simulink model "sm_wheel_loader"  (R2025a)
settings: Solver=ode23t  StartTime=0.0  StopTime=70  RelTol=1e-3  AbsTol=1e-3  EnableMultiTasking=on
PostLoadFcn:
  | sm_wheel_loader_config_impl(bdroot,'Bucket')
StartFcn:
  | tic
StopFcn:
  | Elapsed_Sim_Time = toc;
  | disp(['Elapsed Sim Time = ' num2str(Elapsed_Sim_Time)]);
undefined symbols (not defined in the file or in its folder): HMPST, Ideal, X, Y, Z
libraries: sm_wheel_loader_lib x9, fl_lib x4, sm_lib x3, sdl_lib x2, wheel_loader_contact_lib x2, nesl_utility x1
Description:
  | Wheel Loader with Hydromechanical Power Split Transmission
  | Copyright 2023-2025 The MathWorks, Inc.
settings Model: Creator=ramesh  LastModifiedBy=smiller
settings ConfigSet: Description=|
  | This is the default simulation configuration set.
  | This configuration is used for simulating the model for IK, RBD simulations.
  | This uses variable-step solver.
settings SolverCC: AutoScaleAbsTol=off  AlgebraicLoopSolver=TrustRegion  DecoupledContinuousIntegration=on  MinimalZcImpactIntegration=on
settings DataIOCC: MaxDataPoints=10000  DSMLogging=off  ReturnWorkspaceOutputs=off  SignalLoggingName=logsout_sm_wheel_loader  OutputTimes=[0:0.01:stopTime]
settings OptimizationCC: LifeSpan=inf
settings DebuggingCC: UnconnectedInputMsg=warning  UnconnectedOutputMsg=warning  UnconnectedLineMsg=warning  AllowSymbolicDim=off  SFUnexpectedBacktrackingDiag=warning  SFNoUnconditionalDefaultTransitionDiag=warning  SFExecutionAtInitializationDiag=none  ArithmeticOperatorsInVariantConditions=warning
settings ModelReferenceCC: EnableRefExpFcnMdlSchedulingChecks=on
settings SFSimCC: SimUseLocalCustomCode=off  CustomCodeUndefinedFunction=UseInterfaceOnly
settings RTWCC: RTWUseLocalCustomCode=off  GPUComputeCapability=3.5  DLArmComputeVersion=19.05
settings CodeAppCC: StateflowObjectComments=on
settings GRTTargetCC: TargetLangStandard=C89/C90 (ANSI)
settings ConfigComp: CovMetricSettings=dw  CovSaveCumulativeToWorkspaceVar=on  CovSaveSingleToWorkspaceVar=on  CovExternalEMLEnable=off  CovSFcnEnable=off
settings SimscapeCC: SimscapeLogType=all  SimscapeLogSimulationStatistics=on  SimscapeLogName=simlog_sm_wheel_loader  SimscapeLogLimitData=off  SimscapeLogDataHistory=10000.0
settings DiagnosticsConfigSet: SimMechanicsUnconnectedFramePorts=none  SimMechanicsConflictingReferenceFrames=none
settings ExplorerConfigSet: InternalSimMechanicsExplorerSettings="<ExplorerConfiguration><canonicalview>default</canonicalview><AnimationSetting><BasePlaybackSpeed>1.0</BasePlaybackSpeed><PlaybackSpeedFactor>4.0</PlaybackSpeedFactor></AnimationSetting><TilePanel><TileInfo><Tiles Columns=\"2\" Count=\"3\" Rows=\"2\"><Column Weight=\"0.5\"/><Column Weight=\"0.5\"/><Row Weight=\"0.5\"/><Row Weight=\"0.5\"/><Tile Height=\"2\" Width=\"1\" X=\"0\" Y=\"0\"/><Tile Height=\"1\" Width=\"1\" X=\"1\" Y=\"0\"/><Tile Height=\"1\" Width=\"1\" X=\"1\" Y=\"1\"/></Tiles></TileInfo><SceneInfo><SceneViewer><BGColor><R>1</R><G>1</G><B>1</B></BGColor><Camera><DoPerspective>off</DoPerspective><Position><X>-0.00528186565900144213</X><Y>-2.61761552453344981</Y><Z>10.0638099418932807</Z></Position><Center><X>-0.00528186565900144213</X><Y>-2.61761552453344981</Y><Z>1.2817155600129837</Z></Center><Up><X>0</X><Y>1</Y><Z>-0</Z></Up><ViewLimDist>1</ViewLimDist><YLim>8.29414102564102684</YLim><XLim>9.06400000000000006</XLim></Camera></SceneViewer><SceneViewer><BGColor><R>1</R><G>1</G><B>1</B></BGColor><Camera><DoPerspective>on</DoPerspective><Position><X>1.34928960365821002e-16</X><Y>1.6204999999999985</Y><Z>1.58342999999999989</Z></Position><Center><X>8.83082669489443361e-17</X><Y>0.620499999999998497</Y><Z>1.58343000000000012</Z></Center><Up><X>0</X><Y>0</Y><Z>1</Z></Up><ViewLimDist>1</ViewLimDist><YLim>0.466307658154998583</YLim><XLim>1.0355017035185734</XLim></Camera></SceneViewer><SceneViewer><BGColor><R>1</R><G>1</G><B>1</B></BGColor><Camera><DoPerspective>on</DoPerspective><Position><X>-4.09999999999999964</X><Y>-0.0795000000000013474</Y><Z>1.08343000000000012</Z></Position><Center><X>-3.09999999999999964</X><Y>-0.079500000000001389</Y><Z>1.08343000000000012</Z></Center><Up><X>0</X><Y>0</Y><Z>1</Z></Up><ViewLimDist>1</ViewLimDist><YLim>0.466307658154998583</YLim><XLim>1.0355017035185734</XLim></Camera></SceneViewer></SceneInfo></TilePanel><MechEditorPanel><Cameras><Camera><Id>Camera2</Id><Value><Name>Track_FrameR_DiffR_toR</Name><NativeCamera><PositionTrackingFeature>Wheel_Loader.Vehicle.Frame_Rear.Camera_Frames.Reference_Camera_DiffR_toR.R</PositionTrackingFeature><CenterTrackingFeature>Wheel_Loader.Vehicle.Frame_Rear.Camera_Frames.Reference_Camera_DiffR_toR.R</CenterTrackingFeature><UpVectorTrackingFeature>Wheel_Loader.Vehicle.Frame_Rear.Camera_Frames.Reference_Camera_DiffR_toR.R</UpVectorTrackingFeature><CenterTrackingOrigin>off</CenterTrackingOrigin><CenterTrackingDirection>-Y</CenterTrackingDirection><UpVectorTrackingDirection>+Z</UpVectorTrackingDirection></NativeCamera></Value></Camera><Camera><Id>Camera3</Id><Value><Name>Track_FrameR_FinalDriveRR</Name><NativeCamera><PositionTrackingFeature>Wheel_Loader.Vehicle.Frame_Rear.Camera_Frames.Reference_Camera_FinalDriveRR.R</PositionTrackingFeature><CenterTrackingFeature>Wheel_Loader.Vehicle.Frame_Rear.Camera_Frames.Reference_Camera_FinalDriveRR.R</CenterTrackingFeature><UpVectorTrackingFeature>Wheel_Loader.Vehicle.Frame_Rear.Camera_Frames.Reference_Camera_FinalDriveRR.R</UpVectorTrackingFeature><CenterTrackingOrigin>off</CenterTrackingOrigin><CenterTrackingDirection>-X</CenterTrackingDirection><UpVectorTrackingDirection>+Z</UpVectorTrackingDirection></NativeCamera></Value></Camera><Camera><Id>Camera4</Id><Value><Name>Track_FrameR_Right</Name><NativeCamera><PositionTrackingFeature>Wheel_Loader.Vehicle.Frame_Rear.Camera_Frames.Reference_Camera_Right.R</PositionTrackingFeature><CenterTrackingFeature>Wheel_Loader.Vehicle.Frame_Rear.Camera_Frames.Reference_Camera_Right.R</CenterTrackingFeature><UpVectorTrackingFeature>Wheel_Loader.World_Frame.W</UpVectorTrackingFeature><CenterTrackingOrigin>off</CenterTrackingOrigin><CenterTrackingDirection>-X</CenterTrackingDirection><UpVectorTrackingDirection>+Z</UpVectorTrackingDirection></NativeCamera></Value></Camera><Camera><Id>Camera5</Id><Value><Name>Track_FrameR_Cab</Name><NativeCamera><PositionTrackingFeature>Wheel_Loader.Vehicle.Frame_Rear.Camera_Frames.Reference_Camera_Cab.R</PositionTrackingFeature><CenterTrackingFeature>Wheel_Loader.Vehicle.Frame_Rear.Camera_Frames.Reference_Camera_Cab.R</CenterTrackingFeature><UpVectorTrackingFeature>Wheel_Loader.World_Frame.W</UpVectorTrackingFeature><CenterTrackingOrigin>off</CenterTrackingOrigin><CenterTrackingDirection>+Y</CenterTrackingDirection><UpVectorTrackingDirection>+Z</UpVectorTrackingDirection></NativeCamera></Value></Camera><Camera><Id>Camera6</Id><Value><Name>Track_FrameR_RR</Name><NativeCamera><PositionTrackingFeature>Wheel_Loader.Vehicle.Frame_Rear.Camera_Frames.Reference_Camera_RR.R</PositionTrackingFeature><CenterTrackingFeature>Wheel_Loader.Vehicle.Frame_Rear.Camera_Frames.Reference_Camera_RR.R</CenterTrackingFeature><UpVectorTrackingFeature>Wheel_Loader.World_Frame.W</UpVectorTrackingFeature><CenterTrackingOrigin>off</CenterTrackingOrigin><CenterTrackingDirection>+X</CenterTrackingDirection><UpVectorTrackingDirection>+Z</UpVectorTrackingDirection></NativeCamera></Value></Camera><Camera><Id>Camera7</Id><Value><Name>Track_FrameR_Rear</Name><NativeCamera><PositionTrackingFeature>Wheel_Loader.Vehicle.Frame_Rear.Camera_Frames.Reference_Camera_Rear.R</PositionTrackingFeature><CenterTrackingFeature>Wheel_Loader.Vehicle.Frame_Rear.Camera_Frames.Reference_Camera_Rear.R</CenterTrackingFeature><UpVectorTrackingFeature>Wheel_Loader.World_Frame.W</UpVectorTrackingFeature><CenterTrackingOrigin>off</CenterTrackingOrigin><CenterTrackingDirection>+Y</CenterTrackingDirection><UpVectorTrackingDirection>+Z</UpVectorTrackingDirection></NativeCamera></Value></Camera><Camera><Id>Camera8</Id><Value><Name>Track_FrameF_RR</Name><NativeCamera><PositionTrackingFeature>Wheel_Loader.Vehicle.Frame_Front.Camera_Frames.Reference_Camera_RR.R</PositionTrackingFeature><CenterTrackingFeature>Wheel_Loader.Vehicle.Frame_Front.Camera_Frames.Reference_Camera_RR.R</CenterTrackingFeature><UpVectorTrackingFeature>Wheel_Loader.Vehicle.Frame_Front.Camera_Frames.Reference_Camera_RR.R</UpVectorTrackingFeature><CenterTrackingOrigin>off</CenterTrackingOrigin><CenterTrackingDirection>+X</CenterTrackingDirection><UpVectorTrackingDirection>+Z</UpVectorTrackingDirection></NativeCamera></Value></Camera><Camera><Id>Camera9</Id><Value><Name>Track_FrameF_ImplRR</Name><NativeCamera><PositionTrackingFeature>Wheel_Loader.Vehicle.Frame_Front.Camera_Frames.Reference_Camera_ImplRR.R</PositionTrackingFeature><CenterTrackingFeature>Wheel_Loader.Vehicle.Frame_Front.Camera_Frames.Reference_Camera_ImplRR.R</CenterTrackingFeature><UpVectorTrackingFeature>Wheel_Loader.Vehicle.Frame_Front.Camera_Frames.Reference_Camera_ImplRR.R</UpVectorTrackingFeature><CenterTrackingOrigin>off</CenterTrackingOrigin><CenterTrackingDirection>+X</CenterTrackingDirection><UpVectorTrackingDirection>+Z</UpVectorTrackingDirection></NativeCamera></Value></Camera><Camera><Id>Camera10</Id><Value><Name>Track_FrameF_Roof</Name><NativeCamera><PositionTrackingFeature>Wheel_Loader.Vehicle.Frame_Front.Camera_Frames.Reference_Camera_Roof.R</PositionTrackingFeature><CenterTrackingFeature>Wheel_Loader.Vehicle.Frame_Front.Camera_Frames.Reference_Camera_Roof.R</CenterTrackingFeature><UpVectorTrackingFeature>Wheel_Loader.Vehicle.Frame_Front.Camera_Frames.Reference_Camera_Roof.R</UpVectorTrackingFeature><CenterTrackingOrigin>off</CenterTrackingOrigin><CenterTrackingDirection>+Y</CenterTrackingDirection><UpVectorTrackingDirection>+Z</UpVectorTrackingDirection></NativeCamera></Value></Camera><Camera><Id>Camera11</Id><Value><Name>Track_FrameR_Driveline_RR</Name><NativeCamera><PositionTrackingFeature>Wheel_Loader.Vehicle.Frame_Rear.Camera_Frames.Reference_Camera_Driveline_RR.R</PositionTrackingFeature><CenterTrackingFeature>Wheel_Loader.Vehicle.Frame_Rear.Camera_Frames.Reference_Camera_Driveline_RR.R</CenterTrackingFeature><UpVectorTrackingFeature>Wheel_Loader.Vehicle.Frame_Rear.Camera_Frames.Reference_Camera_Driveline_RR.R</UpVectorTrackingFeature><CenterTrackingOrigin>off</CenterTrackingOrigin><CenterTrackingDirection>+Y</CenterTrackingDirection><UpVectorTrackingDirection>+Z</UpVectorTrackingDirection></NativeCamera></Value></Camera><Camera><Id>Camera12</Id><Value><Name>Track_FrameR_Driveline_Top</Name><NativeCamera><PositionTrackingFeature>Wheel_Loader.Vehicle.Frame_Rear.Camera_Frames.Reference_Camera_Driveline_Top.R</PositionTrackingFeature><CenterTrackingFeature>Wheel_Loader.Vehicle.Frame_Rear.Camera_Frames.Reference_Camera_Driveline_Top.R</CenterTrackingFeature><UpVectorTrackingFeature>Wheel_Loader.Vehicle.Frame_Rear.Camera_Frames.Reference_Camera_Driveline_Top.R</UpVectorTrackingFeature><CenterTrackingOrigin>off</CenterTrackingOrigin><CenterTrackingDirection>-Z</CenterTrackingDirection><UpVectorTrackingDirection>-X</UpVectorTrackingDirection></NativeCamera></Value></Camera><Camera><Id>Camera13</Id><Value><Name>Track_FrameR_Driveline_Top_FixO</Name><NativeCamera><PositionTrackingFeature>Wheel_Loader.Vehicle.Frame_Rear.Camera_Frames.Reference_Camera_Driveline_Top.R</PositionTrackingFeature><CenterTrackingFeature>Wheel_Loader.Vehicle.Frame_Rear.Camera_Frames.Reference_Camera_Driveline_Top.R</CenterTrackingFeature><UpVectorTrackingFeature>Wheel_Loader.World_Frame.W</UpVectorTrackingFeature><CenterTrackingOrigin>off</CenterTrackingOrigin><CenterTrackingDirection>-Z</CenterTrackingDirection><UpVectorTrackingDirection>+X</UpVectorTrackingDirection></NativeCamera></Value></Camera><Camera><Id>Camera14</Id><Value><Name>Track_FrameR_DiffR_toF</Name><NativeCamera><PositionTrackingFeature>Wheel_Loader.Vehicle.Frame_Rear.Camera_Frames.Reference_Camera_DiffR_toF.R</PositionTrackingFeature><CenterTrackingFeature>Wheel_Loader.Vehicle.Frame_Rear.Camera_Frames.Reference_Camera_DiffR_toF.R</CenterTrackingFeature><UpVectorTrackingFeature>Wheel_Loader.Vehicle.Frame_Rear.Camera_Frames.Reference_Camera_DiffR_toF.R</UpVectorTrackingFeature><CenterTrackingOrigin>off</CenterTrackingOrigin><CenterTrackingDirection>-Y</CenterTrackingDirection><UpVectorTrackingDirection>+Z</UpVectorTrackingDirection></NativeCamera></Value></Camera><Camera><Id>Camera15</Id><Value><Name>Track_FrameR_Driveline_Top_Low</Name><NativeCamera><PositionTrackingFeature>Wheel_Loader.Vehicle.Frame_Rear.Camera_Frames.Reference_Camera_Driveline_TopLow.R</PositionTrackingFeature><CenterTrackingFeature>Wheel_Loader.Vehicle.Frame_Rear.Camera_Frames.Reference_Camera_Driveline_TopLow.R</CenterTrackingFeature><UpVectorTrackingFeature>Wheel_Loader.Vehicle.Frame_Rear.Camera_Frames.Reference_Camera_Driveline_TopLow.R</UpVectorTrackingFeature><CenterTrackingOrigin>off</CenterTrackingOrigin><CenterTrackingDirection>-Z</CenterTrackingDirection><UpVectorTrackingDirection>-X</UpVectorTrackingDirection></NativeCamera></Value></Camera><Camera><Id>Camera16</Id><Value><Name>Track_FrameF_LinkageR</Name><NativeCamera><PositionTrackingFeature>Wheel_Loader.Vehicle.Frame_Front.Camera_Frames.Transform_Camera_LinkageR.F</PositionTrackingFeature><CenterTrackingFeature>Wheel_Loader.Vehicle.Frame_Front.Camera_Frames.Transform_Camera_LinkageR.F</CenterTrackingFeature><UpVectorTrackingFeature>Wheel_Loader.Vehicle.Frame_Front.Camera_Frames.Transform_Camera_LinkageR.F</UpVectorTrackingFeature><CenterTrackingOrigin>off</CenterTrackingOrigin><CenterTrackingDirection>-X</CenterTrackingDirection><UpVectorTrackingDirection>+Z</UpVectorTrackingDirection></NativeCamera></Value></Camera><Camera><Id>Camera17</Id><Value><Name>TrackF_WheelFR</Name><NativeCamera><PositionTrackingFeature>Wheel_Loader.Vehicle.Frame_Front.Camera_Frames.Reference_Camera_WhlFR.R</PositionTrackingFeature><CenterTrackingFeature>Wheel_Loader.Vehicle.Frame_Front.Camera_Frames.Reference_Camera_WhlFR.R</CenterTrackingFeature><UpVectorTrackingFeature>Wheel_Loader.World_Frame.W</UpVectorTrackingFeature><CenterTrackingOrigin>off</CenterTrackingOrigin><CenterTrackingDirection>-X</CenterTrackingDirection><UpVectorTrackingDirection>+Z</UpVectorTrackingDirection></NativeCamera></Value></Camera><Camera><Id>Camera18</Id><Value><Name>TrackF_IsoFR</Name><NativeCamera><PositionTrackingFeature>Wheel_Loader.Vehicle.Frame_Front.Camera_Frames.Reference_Camera_IsoFR.R</PositionTrackingFeature><CenterTrackingFeature>Wheel_Loader.Vehicle.Frame_Front.Camera_Frames.Reference_Camera_IsoFR.R</CenterTrackingFeature><UpVectorTrackingFeature>Wheel_Loader.World_Frame.W</UpVectorTrackingFeature><CenterTrackingOrigin>off</CenterTrackingOrigin><CenterTrackingDirection>-X</CenterTrackingDirection><UpVectorTrackingDirection>+Z</UpVectorTrackingDirection></NativeCamera></Value></Camera></Cameras><GfxPanelCameraMap><MapElement CameraMLId=\"Camera5\" GfxPanelIndex=\"1\"/><MapElement CameraMLId=\"Camera4\" GfxPanelIndex=\"2\"/></GfxPanelCameraMap><VideoCreator><PlaybackSpeedRatio>1</PlaybackSpeedRatio><FrameRate>30</FrameRate><VideoFormat>MPEG-4</VideoFormat><FrameSize>auto</FrameSize></VideoCreator></MechEditorPanel></ExplorerConfiguration>"

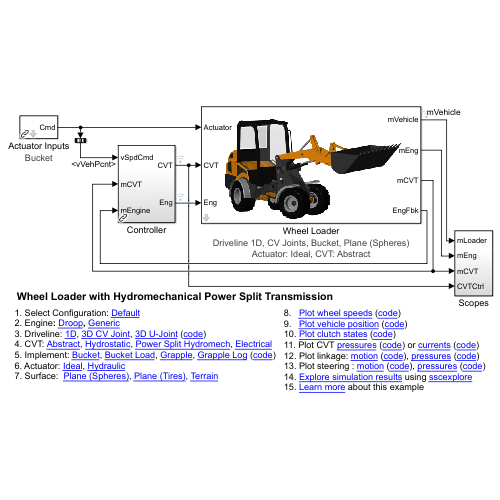
[thumbnail: Simulink's stored preview of the top-level diagram]
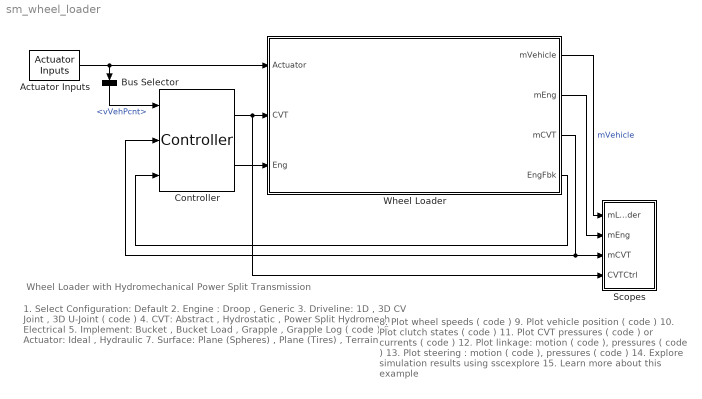
== system sm_wheel_loader ==
  note: Wheel Loader with Hydromechanical Power Split Transmission
  note: 1. Select Configuration: Default
      | 2. Engine : Droop , Generic
      | 3. Driveline: 1D , 3D CV Joint , 3D U-Joint ( code )
      | 4. CVT: Abstract , Hydrostatic , Power Split Hydromech , Electrical
      | 5. Implement: Bucket , Bucket Load , Grapple , Grapple Log ( code )
      | 6. Actuator: Ideal , Hydraulic
      | 7. Surface: Plane (Spheres) , Plane (Tires) , Terrain
  note: 8. Plot wheel speeds ( code )
      | 9. Plot vehicle position ( code )
      | 10. Plot clutch states ( code )
      | 11. Plot CVT pressures ( code ) or currents ( code )
      | 12. Plot linkage: motion ( code ), pressures ( code )
      | 13. Plot steering : motion ( code ), pressures ( code )
      | 14. Explore simulation results using sscexplore
      | 15. Learn more about this example
  Actuator Inputs : sm_wheel_loader_lib/Actuator Inputs  popup_steering=on  popup_linkage=on  popup_impl=Bucket
      settings: AttributesFormatString=%<popup_impl>
  Bus Selector : BusSelector  OutputSignals=Operator.vVehPcnt
  Controller : sm_wheel_loader_lib/Controller  SystemSampleTime=-1  VariantActivationTime=update diagram  EmptyChoice=off  PassThrough=off  PassThroughVariantControl=(default)  EmptyChoiceVariantControl=(default)  AllowFlexibleInterface=on  Latency=0  AutoFrameSizeCalculation=off
      settings: LibrarySourceBlock=sm_wheel_loader_lib/Controller New
  Scopes : Subsystem
  Wheel Loader : Subsystem  mask(Wheel Loader and Load){popup_surface=Plane (Spheres), popup_impl=Bucket, popup_actuator_model=Ideal, popup_cvt=Abstract, popup_engine=Droop, popup_driveline=1D, CV Joints}
      mask prompts: popup_surface "Surface"; popup_impl "Implement"; popup_actuator_model "Actuator Model"; popup_cvt "CVT"; popup_engine "Engine"; popup_driveline "Driveline"
      mask help: Models wheel loader and load. Includes engine, transmission, vehicle and load. Use drop down menus to configure system options.
      mask init:
      | if(popup_surface==1)
      |     set_param([gcb '/Surface'],'LabelModeActiveChoice','Plane')
      |     set_param([gcb '/Vehicle'],'popup_contact','Sphere')
      | elseif(popup_surface==2)
      |     set_param([gcb '/Surface'],'LabelModeActiveChoice','Plane')
      |     set_param([gcb '/Vehicle'],'popup_contact','Tire')
      | elseif(popup_surface==3)
      |     set_param([gcb '/Surface'],'LabelModeActiveChoice','Terrain')
      |     set_param([gcb '/Vehicle'],'popup_contact','Points')
      | end
      | if(popup_impl==1)
      |     set_param([gcb '/Vehicle'],'popup_impl','Bucket')
      |     set_param([gcb '/Vehicle'],'popup_load','None')
      | elseif(popup_impl==2)
      |     set_param([gcb '/Vehicle'],'popup_impl','Bucket')
      |     set_param([gcb '/Vehicle'],'popup_load','Inertia')
      | elseif(popup_impl==3)
      |     set_param([gcb '/Vehicle'],'popup_impl','Grapple')
      |     set_param([gcb '/Vehicle'],'popup_load','None')
      | elseif(popup_impl==4)
      |     set_param([gcb '/Vehicle'],'popup_impl','Grapple')
      |     set_param([gcb '/Vehicle'],'popup_load','Log')
      | end
      | if(popup_cvt==1)
      |     set_param([gcb '/Transmission'],'LabelModeActiveChoice','Abstract')
      | elseif(popup_cvt==2)
      |     set_param([gcb '/Transmission'],'LabelModeActiveChoice','Power_Split_HM')
      | elseif(popup_cvt==3)
      |     set_param([gcb '/Transmission'],'LabelModeActiveChoice','Hydrostatic')
      | elseif(popup_cvt==4)
      |     set_param([gcb '/Transmission'],'LabelModeActiveChoice','Electrical')
      | end
      | if(popup_engine==1)
      |     set_param([gcb '/Engine'],'LabelModeActiveChoice','Droop')
      | else
      |     set_param([gcb '/Engine'],'LabelModeActiveChoice','Generic')
      | end
      | if(popup_driveline==1)
      |     set_param([gcb '/Vehicle'],'popup_driveline_model','Driveline 1D')
      |     set_param([gcb '/Vehicle'],'popup_driveJointF','CV Joint')
      |     set_param([gcb '/Vehicle'],'popup_driveJointR','CV Joint')
      | elseif(popup_driveline==2)
      |     set_param([gcb '/Vehicle'],'popup_driveline_model','Driveline 3D')
      |     set_param([gcb '/Vehicle'],'popup_driveJointF','CV Joint')
      |     set_param([gcb '/Vehicle'],'popup_driveJointR','CV Joint')
      | elseif(popup_driveline==3)
      |     set_param([gcb '/Vehicle'],'popup_driveline_model','Driveline 3D')
      |     set_param([gcb '/Vehicle'],'popup_driveJointF','U Joint')
      |     set_param([gcb '/Vehicle'],'popup_driveJointR','U Joint')
      | end
      settings: AttributesFormatString=|
      | Driveline %<popup_driveline>, %<popup_impl>, %<popup_surface>
      | Actuator: %<popup_actuator_model>, CVT: %<popup_cvt>
      mask TypeOptions popup_surface: Plane (Spheres) | Plane (Tires) | Terrain
      mask TypeOptions popup_impl: Bucket | Bucket Load | Grapple | Grapple Log
      mask TypeOptions popup_actuator_model: Vehicle/popup_actuator_model
      mask TypeOptions popup_cvt: Abstract | Power Split Hydromechanical | Hydrostatic | Electrical
      mask TypeOptions popup_engine: Droop | Generic
      mask TypeOptions popup_driveline: 1D, CV Joints | 3D, CV Joints | 3D, U Joints
      mask Display: image('sm_wheel_loader_vehicle_IMAGE.png');
  wires:
  Wheel Loader/4(EngFbk) -> Controller/3
  Controller/2 -> Wheel Loader/3(Eng)
  Controller/1 -> Scopes/4(CVTCtrl), Wheel Loader/2(CVT)
  Wheel Loader/1(mVehicle) -> Scopes/1(mLoader)  "mVehicle"
  Wheel Loader/2(mEng) -> Scopes/2(mEng)
  Bus Selector/1 -> Controller/1  "<vVehPcnt>"
  Wheel Loader/3(mCVT) -> Scopes/3(mCVT), Controller/2
  Actuator Inputs/1 -> Wheel Loader/1(Actuator), Bus Selector/1

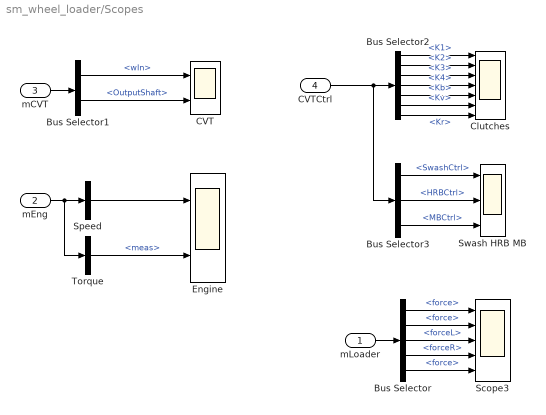
== system sm_wheel_loader/Scopes ==
  mLoader : Inport
  mEng : Inport  Port=2
  mCVT : Inport  Port=3
  CVTCtrl : Inport  Port=4
  Bus Selector : BusSelector  OutputSignals=Linkage.Tilt.force,Linkage.Lift.force,Linkage.Impl.forceL,Linkage.Impl.forceR,Steer.force
  Bus Selector1 : BusSelector  OutputSignals=wIn,OutputShaft
  Bus Selector2 : BusSelector  OutputSignals=K1,K2,K3,K4,Kb,Kv,Kr
  Bus Selector3 : BusSelector  OutputSignals=SwashCtrl,HRBCtrl,MBCtrl
  CVT : Scope  NumInputPorts=2
      settings: ActiveDisplayYMinimum=-1460.02488  ActiveDisplayYMaximum=1460.04785  DataLoggingVariableName=ScopeData4
  Clutches : Scope  NumInputPorts=7
      settings: ActiveDisplayYMinimum=-0.125  ActiveDisplayYMaximum=1.125  DataLoggingVariableName=ScopeData3
  Engine : Scope  NumInputPorts=2
      settings: ActiveDisplayYMinimum=2171.94007  ActiveDisplayYMaximum=2176.05829
  Scope3 : Scope  NumInputPorts=5
      settings: ActiveDisplayYMinimum=-45915.81294  ActiveDisplayYMaximum=93170.95314
  Speed : BusSelector  OutputSignals=w.cmd,w.meas  OutputAsBus=on
  Swash HRB MB : Scope  NumInputPorts=3
      settings: ActiveDisplayYMinimum=-0.96987  ActiveDisplayYMaximum=1.21887  DataLoggingVariableName=ScopeData4
  Torque : BusSelector  OutputSignals=trq.meas
  wires:
  Bus Selector1/1 -> CVT/1  "<wIn>"
  mCVT/1 -> Bus Selector1/1
  Bus Selector2/1 -> Clutches/1  "<K1>"
  CVTCtrl/1 -> Bus Selector3/1, Bus Selector2/1
  Bus Selector3/2 -> Swash HRB MB/2  "<HRBCtrl>"
  Bus Selector2/3 -> Clutches/3  "<K3>"
  Bus Selector2/6 -> Clutches/6  "<Kv>"
  Bus Selector2/2 -> Clutches/2  "<K2>"
  Bus Selector3/1 -> Swash HRB MB/1  "<SwashCtrl>"
  Bus Selector3/3 -> Swash HRB MB/3  "<MBCtrl>"
  Bus Selector2/4 -> Clutches/4  "<K4>"
  Bus Selector2/5 -> Clutches/5  "<Kb>"
  Bus Selector2/7 -> Clutches/7  "<Kr>"
  mEng/1 -> Torque/1, Speed/1
  Speed/1 -> Engine/1
  mLoader/1 -> Bus Selector/1
  Bus Selector/1 -> Scope3/1  "<force>"
  Bus Selector/2 -> Scope3/2  "<force>"
  Torque/1 -> Engine/2  "<meas>"
  Bus Selector/4 -> Scope3/4  "<forceR>"
  Bus Selector/3 -> Scope3/3  "<forceL>"
  Bus Selector/5 -> Scope3/5  "<force>"
  Bus Selector1/2 -> CVT/2  "<OutputShaft>"

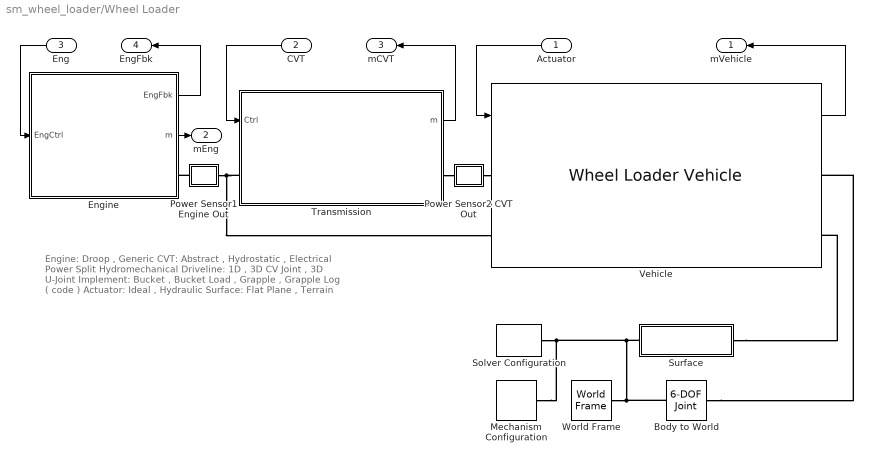
== system sm_wheel_loader/Wheel Loader ==
  note: Engine: Droop , Generic
      | CVT: Abstract , Hydrostatic , Electrical
      | Power Split Hydromechanical
      | Driveline: 1D , 3D CV Joint , 3D U-Joint
      | Implement: Bucket , Bucket Load ,
      | Grapple , Grapple Log ( code )
      | Actuator: Ideal , Hydraulic
      | Surface: Flat Plane , Terrain
  Actuator : Inport
  CVT : Inport  Port=2
  Eng : Inport  Port=3
  Body to World : sm_lib/Joints/6-DOF Joint  JointMode=Normal  CompositeWrenchDir=FollowerOnBase  CompositeWrenchFrame=BaseFrame  SenseConstraintForce=off  SenseConstraintTorque=off  SenseTotalForce=off  SenseTotalTorque=off  PxPositionTargetSpecify=off  PxPositionTargetPriority=High  PxPositionTargetValue=0  PxPositionTargetValueUnits=m  PxVelocityTargetSpecify=off  PxVelocityTargetPriority=High  PxVelocityTargetValue=0  PxVelocityTargetValueUnits=m/s  PxEquilibriumPosition=0  PxEquilibriumPositionUnits=m  PxSpringStiffness=0  PxSpringStiffnessUnits=N/m  PxDampingCoefficient=0  PxDampingCoefficientUnits=N/(m/s)  PxLowerLimitSpecify=off  PxLowerLimitBound=-1  PxLowerLimitBoundUnits=m  PxLowerLimitStiffness=1e6  PxLowerLimitStiffnessUnits=N/m  PxLowerLimitDamping=1e3  PxLowerLimitDampingUnits=N/(m/s)  PxLowerLimitTransitionRegionWidth=1e-4  PxLowerLimitTransitionRegionWidthUnits=m  PxUpperLimitSpecify=off  PxUpperLimitBound=1  PxUpperLimitBoundUnits=m  PxUpperLimitStiffness=1e6  PxUpperLimitStiffnessUnits=N/m  PxUpperLimitDamping=1e3  PxUpperLimitDampingUnits=N/(m/s)  PxUpperLimitTransitionRegionWidth=1e-4  PxUpperLimitTransitionRegionWidthUnits=m  PxTorqueActuationMode=NoTorque  PxMotionActuationMode=ComputedMotion  PxSensePosition=off  PxSenseVelocity=off  PxSenseAcceleration=off  PxSenseTorqueForce=off  PxSenseLowerLimitTorqueForce=off  PxSenseUpperLimitTorqueForce=off  PyPositionTargetSpecify=off  PyPositionTargetPriority=High  PyPositionTargetValue=0  PyPositionTargetValueUnits=m  PyVelocityTargetSpecify=off  PyVelocityTargetPriority=High  PyVelocityTargetValue=0  PyVelocityTargetValueUnits=m/s  PyEquilibriumPosition=0  PyEquilibriumPositionUnits=m  PySpringStiffness=0  PySpringStiffnessUnits=N/m  PyDampingCoefficient=0  PyDampingCoefficientUnits=N/(m/s)  PyLowerLimitSpecify=off  PyLowerLimitBound=-1  PyLowerLimitBoundUnits=m  PyLowerLimitStiffness=1e6  PyLowerLimitStiffnessUnits=N/m  PyLowerLimitDamping=1e3  PyLowerLimitDampingUnits=N/(m/s)  PyLowerLimitTransitionRegionWidth=1e-4  PyLowerLimitTransitionRegionWidthUnits=m  PyUpperLimitSpecify=off  PyUpperLimitBound=1  PyUpperLimitBoundUnits=m  PyUpperLimitStiffness=1e6  PyUpperLimitStiffnessUnits=N/m  PyUpperLimitDamping=1e3  PyUpperLimitDampingUnits=N/(m/s)  PyUpperLimitTransitionRegionWidth=1e-4  PyUpperLimitTransitionRegionWidthUnits=m  PyTorqueActuationMode=NoTorque  PyMotionActuationMode=ComputedMotion  PySensePosition=off  PySenseVelocity=off  PySenseAcceleration=off  PySenseTorqueForce=off  PySenseLowerLimitTorqueForce=off  PySenseUpperLimitTorqueForce=off  PzPositionTargetSpecify=on  PzPositionTargetPriority=High  PzPositionTargetValue=0  PzPositionTargetValueUnits=m  PzVelocityTargetSpecify=off  PzVelocityTargetPriority=High  PzVelocityTargetValue=0  PzVelocityTargetValueUnits=m/s  PzEquilibriumPosition=0  PzEquilibriumPositionUnits=m  PzSpringStiffness=0  PzSpringStiffnessUnits=N/m  PzDampingCoefficient=0  PzDampingCoefficientUnits=N/(m/s)  PzLowerLimitSpecify=off  PzLowerLimitBound=-1  PzLowerLimitBoundUnits=m  PzLowerLimitStiffness=1e6  PzLowerLimitStiffnessUnits=N/m  PzLowerLimitDamping=1e3  PzLowerLimitDampingUnits=N/(m/s)  PzLowerLimitTransitionRegionWidth=1e-4  PzLowerLimitTransitionRegionWidthUnits=m  PzUpperLimitSpecify=off  PzUpperLimitBound=1  PzUpperLimitBoundUnits=m  PzUpperLimitStiffness=1e6  PzUpperLimitStiffnessUnits=N/m  PzUpperLimitDamping=1e3  PzUpperLimitDampingUnits=N/(m/s)  PzUpperLimitTransitionRegionWidth=1e-4  PzUpperLimitTransitionRegionWidthUnits=m  PzTorqueActuationMode=NoTorque  PzMotionActuationMode=ComputedMotion  PzSensePosition=off  PzSenseVelocity=off  PzSenseAcceleration=off  PzSenseTorqueForce=off  PzSenseLowerLimitTorqueForce=off  PzSenseUpperLimitTorqueForce=off  SphPositionTargetSpecify=on  SphPositionTargetPriority=High  SphPositionTargetRotationMethod=StandardAxis  SphPositionTargetFollAlignAxisA=+X  SphPositionTargetBaseAlignAxisA=+Y  SphPositionTargetFollAlignAxisB=+Y  SphPositionTargetBaseAlignAxisB=+Z  SphPositionTargetRotationStandardAxis=+Z  SphPositionTargetRotationAngle=-90  SphPositionTargetRotationAngleUnits=deg  SphPositionTargetRotationArbitraryAxis=[0 0 1]  SphPositionTargetRotationSequenceAxes=FollowerAxes  SphPositionTargetRotationSequence=XYX  SphPositionTargetRotationSequenceAngles=[0 0 0]  SphPositionTargetRotationSequenceAnglesUnits=deg  SphPositionTargetRotationMatrix=[1 0 0; 0 1 0; 0 0 1]  SphPositionTargetQuaternion=[1 0 0 0]  SphVelocityTargetSpecify=off  SphVelocityTargetPriority=High  SphVelocityTargetValue=[0 0 0]  SphVelocityTargetValueUnits=deg/s  SphVelocityTargetInFollowerFrame=on  SphEqPosRotationMethod=None  SphEqPosFollAlignAxisA=+X  SphEqPosBaseAlignAxisA=+Y  SphEqPosFollAlignAxisB=+Y  SphEqPosBaseAlignAxisB=+Z  SphEqPosRotationStandardAxis=+Z  SphEqPosRotationAngle=0.0  SphEqPosRotationAngleUnits=deg  SphEqPosRotationArbitraryAxis=[0 0 1]  SphEqPosRotationSequenceAxes=FollowerAxes  SphEqPosRotationSequence=XYX  SphEqPosRotationSequenceAngles=[0 0 0]  SphEqPosRotationSequenceAnglesUnits=deg  SphEqPosRotationMatrix=[1 0 0; 0 1 0; 0 0 1]  SphEqPosQuaternion=[1 0 0 0]  SphSpringStiffness=0  SphSpringStiffnessUnits=N*m/deg  SphDampingCoefficient=0  SphDampingCoefficientUnits=N*m/(deg/s)  SphLowerLimitSpecify=off  SphLowerLimitBound=15  SphLowerLimitBoundUnits=deg  SphLowerLimitStiffness=1e4  SphLowerLimitStiffnessUnits=N*m/deg  SphLowerLimitDamping=10  SphLowerLimitDampingUnits=N*m/(deg/s)  SphLowerLimitTransitionRegionWidth=0.1  SphLowerLimitTransitionRegionWidthUnits=deg  SphUpperLimitSpecify=off  SphUpperLimitBound=45  SphUpperLimitBoundUnits=deg  SphUpperLimitStiffness=1e4  SphUpperLimitStiffnessUnits=N*m/deg  SphUpperLimitDamping=10  SphUpperLimitDampingUnits=N*m/(deg/s)  SphUpperLimitTransitionRegionWidth=0.1  SphUpperLimitTransitionRegionWidthUnits=deg  SphTorqueActuationMode=NoTorque  SphActuateTorqueX=off  SphActuateTorqueY=off  SphActuateTorqueZ=off  SphActuateTorque=off  SphActuationFrame=BaseFrame  SphSensePosition=off  SphSenseVelocityX=off  SphSenseVelocityY=off  SphSenseVelocityZ=off  SphSenseVelocity=off  SphSenseAccelerationX=off  SphSenseAccelerationY=off  SphSenseAccelerationZ=off  SphSenseAcceleration=off  SphSenseLowerLimitTorqueMag=off  SphSenseUpperLimitTorqueMag=off  SphSensingFrame=BaseFrame
  Engine : Subsystem  Variant=on  VariantControlMode=label  VariantControl=Choice  LabelModeActiveChoice=Droop
      settings: AttributesFormatString=%<LabelModeActiveChoice>
  Mechanism Configuration : sm_lib/Utilities/Mechanism Configuration  UniformGravity=Constant  GravityVector=[0 0 -9.80665]  GravityVectorUnits=m/s^2  LinearizationDelta=0.001  JointModeTransitionNonlinearIterations=2
  Power Sensor1 Engine Out : Subsystem
  Power Sensor2 CVT Out : Subsystem
  Solver Configuration : nesl_utility/Solver Configuration  PhysicalDomain=network_engine_domain  SubClassName=solver  LeftPortType=input  RightPortType=generic  Tones=[]  Harmonics=[]  SimulateNoise=off  Profile=off  UseLocalSampling=off  EnableSwitchedLinearOptims=on  FrequencyDomain=off  UseCCode=off  RelTol=0.001  AbsTol=0.001  MinStep=1e-09  ToWorkspace=off  RevertToSquareIcSolve=off  NumHomotopyIterations=100  PhasorMode=off  PhasorModeNumHarmonics=1  ConsistencySolver=NEWTON_XTOL_AFTER_FTOL  IndexReductionMethod=DerivativeReplacement  DoDC=off  ResidualTolerance=1e-09  ConsistencyTolSource=GLOBAL  ConsistencyAbsTol=0.001  ConsistencyRelTol=0.001  ConsistencyTolFactor=0.001  UseLocalSolver=off  LocalSolverChoice=NE_BACKWARD_EULER_ADVANCER  ResolveIndetEquations=on  FunctionEvalNumThread=1  LocalSolverSampleTime=0.001  DoFixedCost=off  MaxNonlinIter=3  MaxModeIter=2  ComputeImpulses=off  ImpulseIterations=2  LinearAlgebra=auto  LinearAlgebraNumThread=0  EquationFormulation=NE_TIME_EF  DelaysMemoryBudget=1024  AutomaticFiltering=on  FilteringTimeConstant=0.001  PartitionStorageMethod=AS_NEEDED  PartitionMemoryBudget=1024  PartitionMethod=ROBUST  MultibodyUseLocalSolver=off  MultibodyLocalSolverChoice=ODE1  MultibodyLocalSolverSampleTime=0.001
  Surface : Subsystem  Variant=on  VariantControlMode=label  VariantControl=Choice  LabelModeActiveChoice=Plane
  Transmission : Subsystem  Variant=on  VariantControlMode=label  VariantControl=Choice  LabelModeActiveChoice=Abstract
      settings: AttributesFormatString=%<LabelModeActiveChoice>
  Vehicle : sm_wheel_loader_lib/Wheel Loader Vehicle  VariantControl=simVariant == 1  popup_impl=Bucket  popup_actuator_model=Ideal  popup_load=None  popup_driveline_model=Driveline 1D  popup_driveJointF=CV Joint  popup_driveJointR=CV Joint  popup_contact=Sphere
      settings: AttributesFormatString=|
      | %<popup_driveline_model> (F: %<popup_driveJointF>, R: %<popup_driveJointR>), %<popup_contact>
      | %<popup_actuator_model>, %<popup_impl> %<popup_load>
  World Frame : sm_lib/Frames and Transforms/World Frame
  mVehicle : Outport
  mEng : Outport  Port=2
  mCVT : Outport  Port=3
  EngFbk : Outport  Port=4
  wires:
  Engine/1(EngFbk) -> EngFbk/1
  Eng/1 -> Engine/1(EngCtrl)
  Transmission/1(m) -> mCVT/1
  CVT/1 -> Transmission/1(Ctrl)
  Actuator/1 -> Vehicle/1
  Vehicle/1 -> mVehicle/1
  Engine/2(m) -> mEng/1
  connections:
  Transmission/LConn1 -- Vehicle/LConn2 -- Power Sensor1 Engine Out/RConn1
  Solver Configuration/RConn1 -- Surface/LConn1 -- Body to World/LConn1 -- World Frame/RConn1 -- Mechanism Configuration/RConn1
  Body to World/RConn1 -- Vehicle/RConn1
  Surface/RConn1 -- Vehicle/RConn2
  Transmission/RConn1 -- Power Sensor2 CVT Out/LConn1
  Power Sensor1 Engine Out/LConn1 -- Engine/RConn1
  Power Sensor2 CVT Out/RConn1 -- Vehicle/LConn1

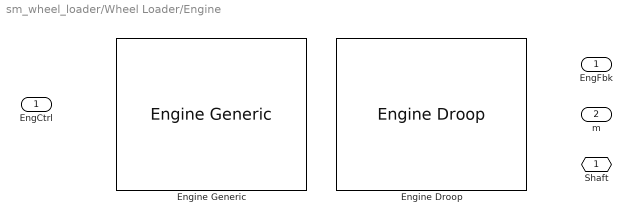
== system sm_wheel_loader/Wheel Loader/Engine ==
  EngCtrl : Inport
  Engine Droop : sm_wheel_loader_lib/Engine Droop  SystemSampleTime=-1  VariantControl=Droop  VariantActivationTime=update diagram  EmptyChoice=off  PassThrough=off  PassThroughVariantControl=(default)  EmptyChoiceVariantControl=(default)  AllowFlexibleInterface=on  Latency=0  AutoFrameSizeCalculation=off
  Engine Generic : sm_wheel_loader_lib/Engine Generic  SystemSampleTime=-1  VariantControl=Generic  VariantActivationTime=update diagram  EmptyChoice=off  PassThrough=off  PassThroughVariantControl=(default)  EmptyChoiceVariantControl=(default)  AllowFlexibleInterface=on  Latency=0  AutoFrameSizeCalculation=off
  Shaft : PMIOPort  Side=Right
  EngFbk : Outport
  m : Outport  Port=2

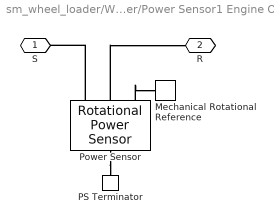
== system sm_wheel_loader/Wheel Loader/Power Sensor1 Engine Out ==
  Mechanical Rotational Reference : fl_lib/Mechanical/Rotational Elements/Mechanical Rotational Reference
  PS Terminator : fl_lib/Physical Signals/Sinks/PS Terminator
  Power Sensor : sdl_lib/Sensors/Rotational Power Sensor  measurement_type=sdl.enum.rotationalPowerSensorType.instantaneous  averaging_period=1 s  max_frequency=1000 Hz  max_speed=1000 rpm
      settings: InternalSimscapePortConfiguration="{\"Bottom\":[],\"Left\":[{\"id\":\"S\",\"label\":\"S\",\"type\":\"foundation.mechanical.rotational.rotational\"},{\"id\":\"R\",\"label\":\"R\",\"type\":\"foundation.mechanical.rotational.rotational\"},{\"id\":\"C\",\"label\":\"C\",\"type\":\"foundation.mechanical.rotational.rotational\"}],\"Right\":[{\"id\":\"P\",\"label\":\"P\",\"type\":\"output\"}],\"Top\":[]}"
  S : PMIOPort  Side=Left
  R : PMIOPort  Port=2  Side=Right
  connections:
  Power Sensor/RConn1 -- PS Terminator/LConn1
  Power Sensor/LConn3 -- Mechanical Rotational Reference/LConn1
  Power Sensor/LConn2 -- R/RConn1
  Power Sensor/LConn1 -- S/RConn1

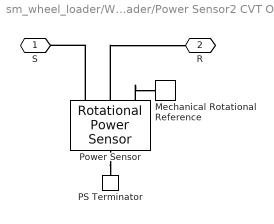
== system sm_wheel_loader/Wheel Loader/Power Sensor2 CVT Out ==
  Mechanical Rotational Reference : fl_lib/Mechanical/Rotational Elements/Mechanical Rotational Reference
  PS Terminator : fl_lib/Physical Signals/Sinks/PS Terminator
  Power Sensor : sdl_lib/Sensors/Rotational Power Sensor  measurement_type=sdl.enum.rotationalPowerSensorType.instantaneous  averaging_period=1 s  max_frequency=1000 Hz  max_speed=1000 rpm
      settings: InternalSimscapePortConfiguration="{\"Bottom\":[],\"Left\":[{\"id\":\"S\",\"label\":\"S\",\"type\":\"foundation.mechanical.rotational.rotational\"},{\"id\":\"R\",\"label\":\"R\",\"type\":\"foundation.mechanical.rotational.rotational\"},{\"id\":\"C\",\"label\":\"C\",\"type\":\"foundation.mechanical.rotational.rotational\"}],\"Right\":[{\"id\":\"P\",\"label\":\"P\",\"type\":\"output\"}],\"Top\":[]}"
  S : PMIOPort  Side=Left
  R : PMIOPort  Port=2  Side=Right
  connections:
  Power Sensor/LConn1 -- S/RConn1
  Power Sensor/LConn2 -- R/RConn1
  Power Sensor/LConn3 -- Mechanical Rotational Reference/LConn1
  Power Sensor/RConn1 -- PS Terminator/LConn1

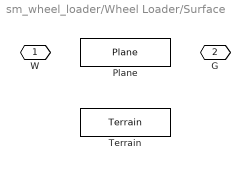
== system sm_wheel_loader/Wheel Loader/Surface ==
  Plane : wheel_loader_contact_lib/Plane  VariantControl=Plane
  Terrain : wheel_loader_contact_lib/Terrain  VariantControl=Terrain
  W : PMIOPort  Side=Left
  G : PMIOPort  Port=2  Side=Right

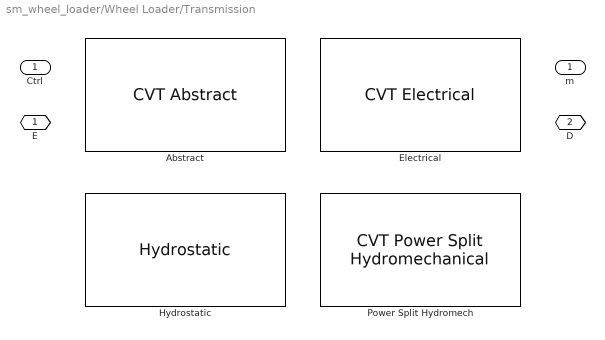
== system sm_wheel_loader/Wheel Loader/Transmission ==
  Ctrl : Inport
  Abstract : sm_wheel_loader_lib/CVT Abstract  VariantControl=Abstract  dShaftE=HMPST.AbstractCVT.dInput  dShaftD=HMPST.AbstractCVT.dOutput  k=HMPST.AbstractCVT.kCompliance  d=HMPST.AbstractCVT.dCompliance
  Electrical : sm_wheel_loader_lib/CVT Electrical  VariantControl=Electrical
  Hydrostatic : sm_wheel_loader_lib/Hydrostatic  SystemSampleTime=-1  VariantControl=Hydrostatic  VariantActivationTime=update diagram  EmptyChoice=off  PassThrough=off  PassThroughVariantControl=(default)  EmptyChoiceVariantControl=(default)  AllowFlexibleInterface=on  Latency=0  AutoFrameSizeCalculation=off
  Power Split Hydromech : sm_wheel_loader_lib/CVT Power Split Hydromechanical  SystemSampleTime=-1  VariantControl=Power_Split_HM  VariantActivationTime=update diagram  EmptyChoice=off  PassThrough=off  PassThroughVariantControl=(default)  EmptyChoiceVariantControl=(default)  AllowFlexibleInterface=on  Latency=0  AutoFrameSizeCalculation=off
      settings: LibrarySourceBlock=sm_wheel_loader_lib/CVT Powersplit Hydromechanical
  E : PMIOPort  Side=Left
  D : PMIOPort  Port=2  Side=Right
  m : Outport
